simulink model "TF02_pro_Test"  (R2026b)
settings: Solver=VariableStepAuto
undefined symbols (not defined in the file or in its folder): Lidar_1, Lidar_2
libraries: aerolibutil x4, sharedutil x1
settings Model: Creator=11and  LastModifiedBy=11and

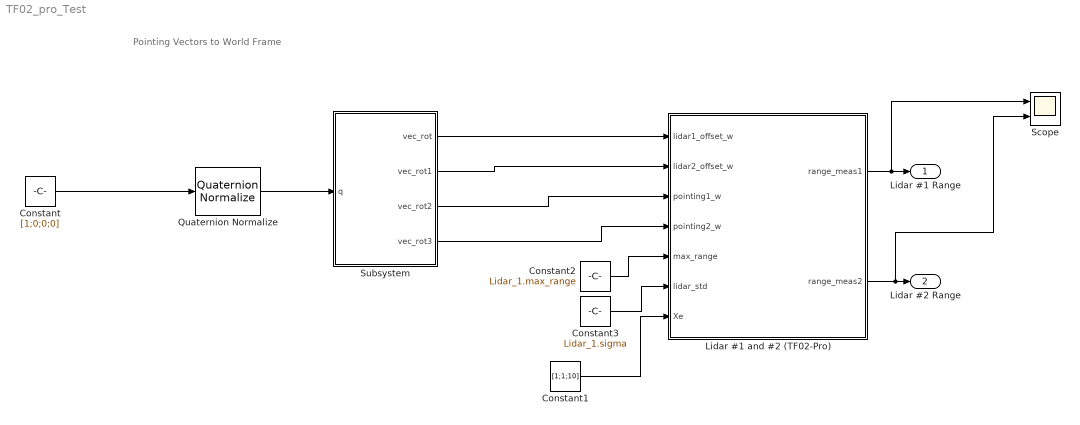
== system TF02_pro_Test ==
  note: Pointing Vectors to World Frame
  Constant : Constant  Value=[1;0;0;0]
  Constant1 : Constant  Value=[1;1;10]
  Constant2 : Constant  Value=Lidar_1.max_range
  Constant3 : Constant  Value=Lidar_1.sigma
  Lidar #1 and #2 (TF02-Pro) : MATLAB Function  TreatAsAtomicUnit=on  SystemSampleTime=1/Lidar_1.sample_rate
  Quaternion Normalize : sharedutil/Quaternion Normalize  aMode=aMode
  Scope : Scope  NumInputPorts=2
      settings: ActiveDisplayYMinimum=17.310379470929728  ActiveDisplayYMaximum=17.650901207713019
  Subsystem : Subsystem
  Lidar #1 Range : Outport
  Lidar #2 Range : Outport  Port=2
  wires:
  Lidar #1 and #2 (TF02-Pro)/2(range_meas2) -> Scope/2, Lidar #2 Range/1
  Subsystem/3(vec_rot2) -> Lidar #1 and #2 (TF02-Pro)/3(pointing1_w)
  Quaternion Normalize/1 -> Subsystem/1(q)
  Constant2/1 -> Lidar #1 and #2 (TF02-Pro)/5(max_range)
  Subsystem/4(vec_rot3) -> Lidar #1 and #2 (TF02-Pro)/4(pointing2_w)
  Subsystem/1(vec_rot) -> Lidar #1 and #2 (TF02-Pro)/1(lidar1_offset_w)
  Constant3/1 -> Lidar #1 and #2 (TF02-Pro)/6(lidar_std)
  Lidar #1 and #2 (TF02-Pro)/1(range_meas1) -> Scope/1, Lidar #1 Range/1
  Constant/1 -> Quaternion Normalize/1
  Subsystem/2(vec_rot1) -> Lidar #1 and #2 (TF02-Pro)/2(lidar2_offset_w)
  Constant1/1 -> Lidar #1 and #2 (TF02-Pro)/7(Xe)

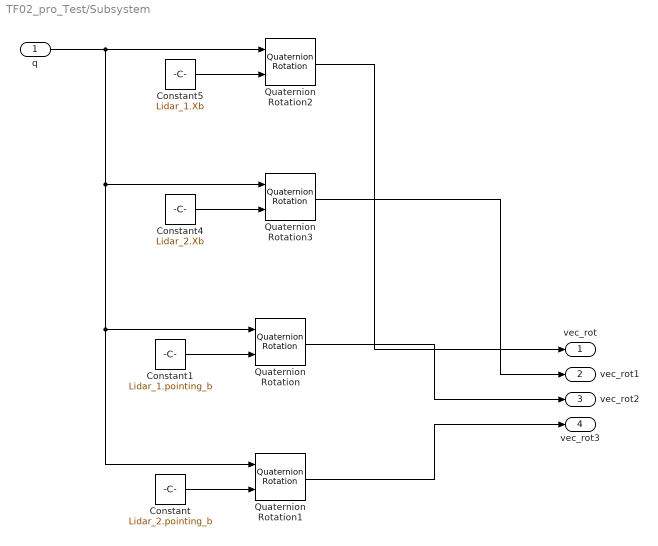
== system TF02_pro_Test/Subsystem ==
  q : Inport
  Constant : Constant  Value=Lidar_2.pointing_b
  Constant1 : Constant  Value=Lidar_1.pointing_b
  Constant4 : Constant  Value=Lidar_2.Xb
  Constant5 : Constant  Value=Lidar_1.Xb
  Quaternion Rotation{,1..3} (4 alike) : aerolibutil/Quaternion Rotation
  vec_rot : Outport
  vec_rot1 : Outport  Port=2
  vec_rot2 : Outport  Port=3
  vec_rot3 : Outport  Port=4
  wires:
  q/1 -> Quaternion Rotation1/1, Quaternion Rotation/1, Quaternion Rotation3/1, Quaternion Rotation2/1
  Constant/1 -> Quaternion Rotation1/2
  Constant5/1 -> Quaternion Rotation2/2
  Quaternion Rotation2/1 -> vec_rot/1
  Constant4/1 -> Quaternion Rotation3/2
  Quaternion Rotation/1 -> vec_rot2/1
  Quaternion Rotation3/1 -> vec_rot1/1
  Constant1/1 -> Quaternion Rotation/2
  Quaternion Rotation1/1 -> vec_rot3/1

== matlab function TF02_pro_Test/Lidar #1 and #2 (TF02-Pro) ==
  data: lidar1_offset_w input; lidar2_offset_w input; range_meas1 output; range_meas2 output; pointing1_w input; pointing2_w input; max_range input; lidar_std input; Xe input
function [range_meas1, range_meas2]= fcn(lidar1_offset_w, lidar2_offset_w, pointing1_w, pointing2_w, max_range, lidar_std, Xe)
% lidar_offset_w = lidar offset from Xe, [x_w, y_w, z_w]
% pointing = inertial lidar pointing vector
% max_range = maximum rangefinder depth, m
% lidar_std = standard deviation of lidar data
% Xe = vehicle CG position in world frame


% ground is flat and at inertial z = 0 m
z_ground = 0;

% add sensor cg offset to cg position to get world position
lidar1_pos_w = lidar1_offset_w + Xe;
lidar2_pos_w = lidar2_offset_w + Xe;

% normalize
pointing1_w_unit = pointing1_w/norm(pointing1_w);
pointing2_w_unit = pointing2_w/norm(pointing2_w);

% angle to horizontal = angle to ground
ang1 = (pointing1_w_unit(3)); % sine of angle b/w lidar pointing and horizontal
ang2 = (pointing2_w_unit(3));


%% lidar 1
if abs(sin(ang1)) < 1e-6
    % Beam is parallel to the ground -- never intersects
    range_meas1 = max_range;
else
    t = (z_ground+lidar1_pos_w(3))/ang1;
    if t <= 0 || t > max_range
        % Ground is behind the beam, or intersection is beyond sensor range
        range_meas1 = max_range;      % or NaN, depending on how your estimator handles no-return
    else
        noise = randn(1)*(lidar_std);
        range_meas1 = t +  noise;
    end
end

%% lidar 2
if abs(sin(ang2)) < 1e-6
    % Beam is parallel to the ground -- never intersects
    range_meas2 = max_range;
else
    t = (z_ground+lidar2_pos_w(3))/ang2;
    if t <= 0 || t > max_range
        % Ground is behind the beam, or intersection is beyond sensor range
        range_meas2 = max_range;      % or NaN, depending on how your estimator handles no-return
    else
        noise = randn(1)*(lidar_std);
        range_meas2 = t +  noise;
    end
end
